simulink model "regulator_P"  (R2026b)
settings: Solver=VariableStepAuto  StopTime=300
libraries: fuzblock x1
settings Model: Creator=blajm  LastModifiedBy=blajm

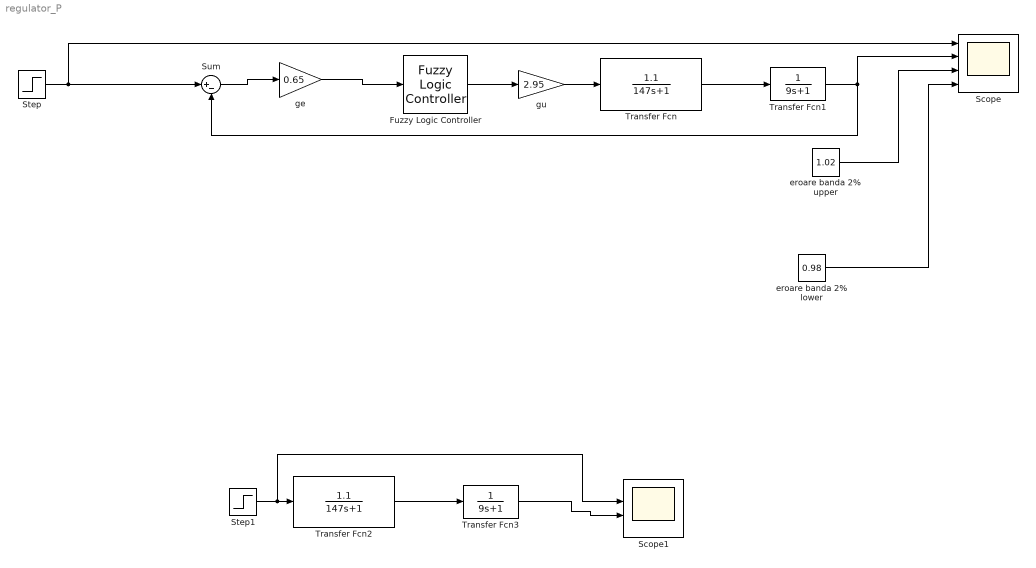
== system regulator_P ==
  Fuzzy Logic Controller : fuzblock/Fuzzy Logic  Controller  FIS=Regulator_Proportional1  OutputSampleNumber=101  DataType=double  UseLookupTable=off  NumBreakpoints=10  FuzzifiedInputs=off  RuleFiringStrengths=off  RuleOutputs=off  AggregatedOutputs=off  SimulateUsing=Interpreted execution  OutOfRangeInputValueMessage=warning  NoRuleFiredMessage=warning  EmptyOutputFuzzySetMessage=warning
  Scope : Scope  NumInputPorts=4
      settings: ActiveDisplayYMinimum=-0.12749999999999997  ActiveDisplayYMaximum=1.1475
  Scope1 : Scope  NumInputPorts=4
      settings: ActiveDisplayYMinimum=-0.13733620105167541  ActiveDisplayYMaximum=1.2360258094650789
  Step : Step  SampleTime=0
  Step1 : Step  SampleTime=0
  Sum : Sum  Inputs=|+-
  Transfer Fcn : TransferFcn  Numerator=[1.1]  Denominator=[147 1]
  Transfer Fcn1 : TransferFcn  Denominator=[9 1]
  Transfer Fcn2 : TransferFcn  Numerator=[1.1]  Denominator=[147 1]
  Transfer Fcn3 : TransferFcn  Denominator=[9 1]
  eroare banda 2% lower : Constant  Value=0.98
  eroare banda 2% upper : Constant  Value=1.02
  ge : Gain  Gain=0.65
  gu : Gain  Gain=2.95
  wires:
  Step/1 -> Scope/1, Sum/1
  Sum/1 -> ge/1
  Fuzzy Logic Controller/1 -> gu/1
  gu/1 -> Transfer Fcn/1
  Transfer Fcn/1 -> Transfer Fcn1/1
  Transfer Fcn1/1 -> Sum/2, Scope/2
  ge/1 -> Fuzzy Logic Controller/1
  eroare banda 2% upper/1 -> Scope/3
  eroare banda 2% lower/1 -> Scope/4
  Transfer Fcn2/1 -> Transfer Fcn3/1
  Step1/1 -> Scope1/2, Transfer Fcn2/1
  Transfer Fcn3/1 -> Scope1/3
